simulink model "PMSMBridgePlantTest"  (R2026b)
settings: Solver=FixedStepDiscrete  StopTime=bridgeTestCfg.Duration  FixedStep=bridgeCfg.Ts
PostLoadFcn:
  | addpath(fullfile(fileparts(get_param(bdroot,'FileName')),'..','build_process'));initialize_bridge_test(bdroot);
model workspace (MAT data in the model file):
  bridgeCfg.Rs = 0.5
  bridgeCfg.Ld = 0.001
  bridgeCfg.Lq = 0.0012
  bridgeCfg.Flux = 0.035
  bridgeCfg.PolePairs = 4
  bridgeCfg.J = 0.0005
  bridgeCfg.B = 0.0001
  bridgeCfg.Id0 = 0
  bridgeCfg.Iq0 = 0
  bridgeCfg.Speed0 = 80
  bridgeCfg.Position0 = 0.1
  bridgeCfg.Ts = 5e-06
  bridgeCfg.Vdc = 48
  bridgeCfg.DiodeVf = 0.7
  bridgeCfg.DiodeRon = 0.01
  bridgeCfg.MechanicalEnabled = 1
  bridgeCfg.CurrentTolerance = 1e-09
  bridgeCfg.VoltageTolerance = 1e-08
  bridgeCfg.MaxCurrent = 200
  bridgeCfg.MaxSpeed = 1000
  bridgeCfg.MaxAngleStep = 0.1
  bridgeCfg.State0 = [0; 0; 80; 0.1]
  bridgeCfg.Vector = [5e-06; 0.5; 0.001; 0.0012; 0.035; 4; 0.0005; 0.0001; 48; 0.7; 0.01; 1; 1e-09; 1e-08; 200; 1000; 0.1]
  bridgeStim.time = [0 5e-06 1e-05 1.5e-05 2e-05 2.5e-05 3e-05 3.5e-05 4e-05 4.5e-05 5e-05 5.5e-05 ... (12001 elements, 12001x1)]
  bridgeStim.signals.values = [0.5 0.5 0.5 0.5 0.5 0.5 0.5 0.5 0.5 0.5 0.5 0.5 ... (60005 elements, 12001x5)]
  bridgeStim.signals.dimensions = 5
  bridgeTestCfg.Duration = 0.06
  bridgeTestCfg.ModeTimes = [0 0.015 0.025]
  bridgeTestCfg.ModeValues = [0 2 0]
  bridgeTestCfg.Duty = [0.5 0.5 0.5]
  bridgeTestCfg.LoadTorque = 0
libraries: PMSMBridgePlant x1
settings Model: Creator=24322  LastModifiedBy=24322

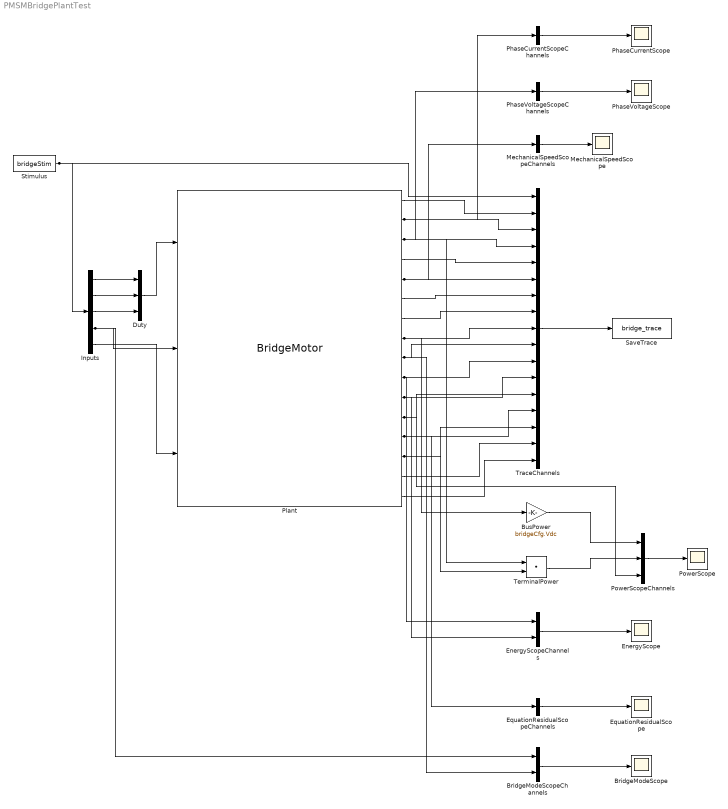
== system PMSMBridgePlantTest ==
  BridgeModeScope : Scope
  BridgeModeScopeChannels : Mux  Inputs=2
  BusPower : Gain  Gain=bridgeCfg.Vdc
  Duty : Mux  Inputs=3
  EnergyScope : Scope
  EnergyScopeChannels : Mux  Inputs=2
  EquationResidualScope : Scope
  EquationResidualScopeChannels : Mux  Inputs=1
  Inputs : Demux  Outputs=5
  MechanicalSpeedScope : Scope
  MechanicalSpeedScopeChannels : Mux  Inputs=1
  PhaseCurrentScope : Scope
  PhaseCurrentScopeChannels : Mux  Inputs=1
  PhaseVoltageScope : Scope
  PhaseVoltageScopeChannels : Mux  Inputs=1
  Plant : PMSMBridgePlant/BridgeMotor  cfg=bridgeCfg
  PowerScope : Scope
  PowerScopeChannels : Mux  Inputs=3
  SaveTrace : ToWorkspace  VariableName=bridge_trace  SaveFormat=Structure With Time  SampleTime=-1
  Stimulus : FromWorkspace  VariableName=bridgeStim  SampleTime=bridgeCfg.Ts  Interpolate=off  OutputAfterFinalValue=Holding final value
  TerminalPower : DotProduct  OutDataTypeStr=Inherit: Inherit via internal rule
  TraceChannels : Mux  Inputs=17
  wires:
  EquationResidualScopeChannels/1 -> EquationResidualScope/1
  EnergyScopeChannels/1 -> EnergyScope/1
  MechanicalSpeedScopeChannels/1 -> MechanicalSpeedScope/1
  PhaseVoltageScopeChannels/1 -> PhaseVoltageScope/1
  PhaseCurrentScopeChannels/1 -> PhaseCurrentScope/1
  Plant/16 -> TraceChannels/17
  Plant/15 -> TraceChannels/16
  Plant/13 -> TraceChannels/14, EquationResidualScopeChannels/1
  Plant/11 -> TraceChannels/12, EnergyScopeChannels/2
  Plant/10 -> TraceChannels/11, EnergyScopeChannels/1
  Plant/7 -> TraceChannels/8
  Plant/6 -> TraceChannels/7
  Plant/5 -> TraceChannels/6, MechanicalSpeedScopeChannels/1
  Plant/4 -> TraceChannels/5
  Plant/2 -> TraceChannels/3, PhaseCurrentScopeChannels/1
  Plant/1 -> TraceChannels/2
  Inputs/3 -> Duty/3
  Inputs/2 -> Duty/2
  Inputs/1 -> Duty/1
  Plant/14 -> TerminalPower/2, TraceChannels/15
  Plant/3 -> TraceChannels/4, TerminalPower/1, PhaseVoltageScopeChannels/1
  Plant/8 -> BusPower/1, TraceChannels/9
  TraceChannels/1 -> SaveTrace/1
  Inputs/5 -> Plant/3
  Duty/1 -> Plant/1
  Stimulus/1 -> Inputs/1, TraceChannels/1
  Inputs/4 -> BridgeModeScopeChannels/1, Plant/2
  Plant/9 -> BridgeModeScopeChannels/2, TraceChannels/10
  Plant/12 -> PowerScopeChannels/3, TraceChannels/13
  PowerScopeChannels/1 -> PowerScope/1
  BusPower/1 -> PowerScopeChannels/1
  TerminalPower/1 -> PowerScopeChannels/2
  BridgeModeScopeChannels/1 -> BridgeModeScope/1
